simulink model "Lab1_Vertical"  (R2026b)
settings: Solver=VariableStepAuto  StopTime=2  MaxStep=0.01  RelTol=1e-6  AbsTol=1e-8
values from neighbouring files (symbols this model uses):
  g = 9.81    [lab1_parameters.m]
  m = m_nom    (= 1.965)    [lab1_parameters.m]
  T_cmd = T_hover    (= 19.27665)    [lab1_parameters.m]
  w0 = 0.40    (= 0.4)    [lab1_parameters.m]
  z0 = 0    [lab1_parameters.m]
settings Model: Creator=nicholas  LastModifiedBy=nicholas

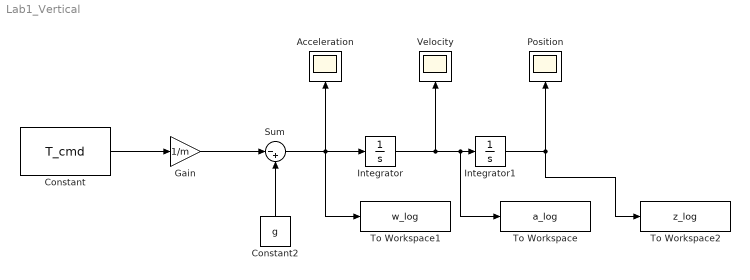
== system Lab1_Vertical ==
  Acceleration : Scope
      settings: ActiveDisplayYMinimum=-5.3753515600036126  ActiveDisplayYMaximum=12.339378087246306
  Constant : Constant  Value=T_cmd
  Constant2 : Constant  Value=g
  Gain : Gain  Gain=1/m
  Integrator : Integrator  InitialCondition=w0
  Integrator1 : Integrator  InitialCondition=z0
  Position : Scope
      settings: ActiveDisplayYMinimum=-19.267779598115222  ActiveDisplayYMaximum=20.84878561855405
  Sum : Sum  Inputs=|-+
  To Workspace : ToWorkspace  VariableName=a_log  SaveFormat=Timeseries  SampleTime=-1
  To Workspace1 : ToWorkspace  VariableName=w_log  SaveFormat=Timeseries  SampleTime=-1
  To Workspace2 : ToWorkspace  VariableName=z_log  SaveFormat=Timeseries  SampleTime=-1
  Velocity : Scope
      settings: ActiveDisplayYMinimum=-2.6471811879671971  ActiveDisplayYMaximum=10.594796302006996  DataLoggingVariableName=ScopeData2
  wires:
  Constant/1 -> Gain/1
  Gain/1 -> Sum/1
  Constant2/1 -> Sum/2
  Sum/1 -> To Workspace1/1, Integrator/1, Acceleration/1
  Integrator/1 -> To Workspace/1, Integrator1/1, Velocity/1
  Integrator1/1 -> To Workspace2/1, Position/1
